simulink model "turbo_controller"  (R2025a)
settings: Solver=FixedStepAuto  StartTime=0.0  StopTime=inf  FixedStep=0.001  RelTol=1e-3
PostLoadFcn:
  | % 自动定位同目录CubeMX文件；不需要外部初始化脚本。
  | codertarget.data.setParameterValue('turbo_controller','STM32CubeMX.ProjectFile',fullfile(fileparts(get_param('turbo_controller','FileName')),'turbo_f407.ioc'));
InitFcn:
  | % 中文说明：按原控制器字段与类型创建三组接口总线；控制参数已内嵌。
  | tc_names=["EValve_Cycle" "EValve_Open" "Eblast_Cycle" "Eblast_Open" "Motor_Cycle" "Motor_Open" "EValve_Enable" "Eblast_Enable" "Motor_Enable" "SWO_Firework" "SWO_BleedAir" "EngineState" "Flag_ECUReset_Clear" "Flag_ECUReset_Save" "Flag_Reset_Enable" "Accelerator" "Nc_dem" "Nc"]; tc_types=["uint16" "uint16" "uint16" "uint16" "uint16" "uint16" "uint8" "uint8" "uint8" "uint8" "uint8" "uint8" "uint8" "uint8" "uint8" "single" "single" "single"];
  | for tc_k=1:numel(tc_names)
  |  tc_e(tc_k)=Simulink.BusElement; tc_e(tc_k).Name=char(tc_names(tc_k)); tc_e(tc_k).DataType=char(tc_types(tc_k));
  | end
  | EngineControl_Out=Simulink.Bus; EngineControl_Out.DataScope='Exported'; EngineControl_Out.Elements=tc_e;
  | clear tc_e tc_names tc_types tc_k
  | tc_names=["savedata1" "savedata2" "savedata3" "savedata4" "savedata5" "savedata6" "savedata7" "savedata8" "savedata9" "savedata10" "savedata11" "savedata12" "savedata13" "savedata14" "savedata15" "savedata16" "savedata17" "savedata18" "savedata19" "savedata20" "savedata21" "savedata22" "savedata23" "savedata24" "savedata25"]; tc_types=["single" "single" "single" "single" "single" "single" "single" "single" "single" "single" "single" "single" "single" "single" "single" "single" "single" "single" "single" "single" "single" "single" "single" "single" "single"];
  | for tc_k=1:numel(tc_names)
  |  tc_e(tc_k)=Simulink.BusElement; tc_e(tc_k).Name=char(tc_names(tc_k)); tc_e(tc_k).DataType=char(tc_types(tc_k));
  | end
  | SaveData_Out=Simulink.Bus; SaveData_Out.DataScope='Exported'; SaveData_Out.Elements=tc_e;
  | clear tc_e tc_names tc_types tc_k
  | tc_names=["senddata1" "senddata2" "senddata3" "senddata4" "senddata5" "senddata6" "senddata7" "senddata8" "senddata9" "senddata10" "senddata11" "senddata12" "senddata13" "senddata14" "senddata15" "senddata16" "senddata17" "senddata18" "senddata19" "senddata20" "senddata21" "senddata22" "senddata23" "senddata24" "senddata25" "senddata26" "senddata27" "senddata28" "senddata29"]; tc_types=["uint8" "uint8" "uint8" "uint8" "uint8" "uint8" "uint8" "uint8" "uint8" "uint8" "uint8" "uint8" "uint8" "uint8" "uint8" "uint8" "uint8" "uint8" "uint8" "uint8" "uint8" "uint8" "uint8" "uint8" "uint8" "uint8" "uint8" "uint8" "uint8"];
  | for tc_k=1:numel(tc_names)
  |  tc_e(tc_k)=Simulink.BusElement; tc_e(tc_k).Name=char(tc_names(tc_k)); tc_e(tc_k).DataType=char(tc_types(tc_k));
  | end
  | SendData_Out=Simulink.Bus; SendData_Out.DataScope='Exported'; SendData_Out.Elements=tc_e;
  | clear tc_e tc_names tc_types tc_k
  | 
  | % 以下为接口中文说明；只设置描述，不改变数值或数据类型。
  | EngineControl_Out.Description='执行控制输出（阀、电机、点火、状态及复位请求）';
  | tc_cn=["EValve_Cycle（主油阀周期计数（每计数2毫秒））" "EValve_Open（主油阀开通计数（每计数2毫秒））" "Eblast_Cycle（副油阀周期计数（每计数2毫秒））" "Eblast_Open（副油阀开通计数（每计数2毫秒））" "Motor_Cycle（起动电机周期计数）" "Motor_Open（起动电机开通计数）" "EValve_Enable（主油阀驱动使能）" "Eblast_Enable（副油阀驱动使能）" "Motor_Enable（起动电机使能）" "SWO_Firework（点火器使能（1开））" "SWO_BleedAir（引气阀使能（1开））" "EngineState（发动机状态）" "Flag_ECUReset_Clear（清除复位恢复状态请求）" "Flag_ECUReset_Save（保存复位恢复数据请求）" "Flag_Reset_Enable（处理器软件复位请求）" "Accelerator（油门／油泵给定控制量）" "Nc_dem（控制目标转速）" "Nc（发动机反馈转速（转每分））"];
  | tc_elements=EngineControl_Out.Elements;
  | for tc_k=1:numel(tc_cn)
  |  tc_elements(tc_k).Description=char(tc_cn(tc_k));
  | end
  | EngineControl_Out.Elements=tc_elements;
  | clear tc_cn tc_elements tc_k
  | SaveData_Out.Description='25项运行记录；字段含义按当前模型数据来源解释';
  | tc_cn=["savedata1（指令回显记录）" "savedata2（入口总温记录（℃））" "savedata3（电源电压记录）" "savedata4（排气温度记录（℃））" "savedata5（标定燃油压力记录）" "savedata6（副油阀占空比记录（％））" "savedata7（主油阀占空比记录（％））" "savedata8（温度修正转速记录）" "savedata9（开关输出及反馈位域）" "savedata10（物理转速记录）" "savedata11（油泵目标给定原始值）" "savedata12（起动电机占空比记录（％））" "savedata13（发动机状态码记录）" "savedata14（故障告警位域记录）" "savedata15（模型记录帧序号）" "savedata16（处理器温度记录（℃））" "savedata17（装订转速记录（沿用旧电源字段名））" "savedata18（导航高度记录）" "savedata19（飞行空速记录）" "savedata20（主阀旧记录位（恒零保留））" "savedata21（第21项保留记录（恒零））" "savedata22（保留记录项22）" "savedata23（保留记录项23）" "savedata24（保留记录项24）" "savedata25（保留记录项25）"];
  | tc_elements=SaveData_Out.Elements;
  | for tc_k=1:numel(tc_cn)
  |  tc_elements(tc_k).Description=char(tc_cn(tc_k));
  | end
  | SaveData_Out.Elements=tc_elements;
  | clear tc_cn tc_elements tc_k
  | SendData_Out.Description='29字段回传及外设命令接口；板端上位机帧只取第3至27字段';
  | tc_cn=["senddata1（回传发送允许标志（不直接上线路））" "senddata2（回传载荷长度25字节）" "senddata3（回传指令回显字节）" "senddata4（总温编码字节（℃＋80））" "senddata5（电源电压编码字节）" "senddata6（排温编码高字节）" "senddata7（排温编码低字节）" "senddata8（燃油压力编码高字节）" "senddata9（燃油压力编码低字节）" "senddata10（副油阀占空比字节（％））" "senddata11（主油阀占空比字节（％））" "senddata12（修正转速编码高字节）" "senddata13（修正转速编码低字节）" "senddata14（驱动及反馈状态位域）" "senddata15（物理转速编码高字节）" "senddata16（物理转速编码低字节）" "senddata17（油泵目标给定高字节（串口二使用））" "senddata18（油泵目标给定低字节（串口二使用））" "senddata19（起动电机占空比命令（串口一使用））" "senddata20（发动机状态码字节）" "senddata21（故障告警位域字节）" "senddata22（帧序号占位（板端另行填写））" "senddata23（处理器温度编码（℃＋50））" "senddata24（控制目标转速编码高字节）" "senddata25（控制目标转速编码低字节）" "senddata26（占位字节（板端改填实测泵速高字节））" "senddata27（占位字节（板端改填实测泵速低字节））" "senddata28（装订转速高字节（本板未发送））" "senddata29（装订转速低字节（本板未发送））"];
  | tc_elements=SendData_Out.Elements;
  | for tc_k=1:numel(tc_cn)
  |  tc_elements(tc_k).Description=char(tc_cn(tc_k));
  | end
  | SendData_Out.Elements=tc_elements;
  | clear tc_cn tc_elements tc_k
  | 
  | 
  | % FRAM模块化事务：接口类型和上电初始状态，随模型保存，无外部初始化文件。
  | clear FM_elements
  | FM_elements(1)=Simulink.BusElement;FM_elements(1).Name='phase';FM_elements(1).DataType='uint8';FM_elements(1).Dimensions=[1 1];FM_elements(1).Description='phase（当前事务阶段）';
  | FM_elements(2)=Simulink.BusElement;FM_elements(2).Name='a';FM_elements(2).DataType='uint8';FM_elements(2).Dimensions=[64 1];FM_elements(2).Description='a（启动时缓存的首区64字节）';
  | FM_elements(3)=Simulink.BusElement;FM_elements(3).Name='active';FM_elements(3).DataType='uint16';FM_elements(3).Dimensions=[1 1];FM_elements(3).Description='active（当前有效记录区地址）';
  | FM_elements(4)=Simulink.BusElement;FM_elements(4).Name='generation';FM_elements(4).DataType='uint32';FM_elements(4).Dimensions=[1 1];FM_elements(4).Description='generation（当前有效记录代号）';
  | FM_elements(5)=Simulink.BusElement;FM_elements(5).Name='record';FM_elements(5).DataType='uint8';FM_elements(5).Dimensions=[64 1];FM_elements(5).Description='record（本次冻结的待写记录）';
  | FM_elements(6)=Simulink.BusElement;FM_elements(6).Name='addr';FM_elements(6).DataType='uint16';FM_elements(6).Dimensions=[1 1];FM_elements(6).Description='addr（本次备用写入地址）';
  | FM_elements(7)=Simulink.BusElement;FM_elements(7).Name='lastSave';FM_elements(7).DataType='single';FM_elements(7).Dimensions=[1 1];FM_elements(7).Description='lastSave（上次开始保存的秒数）';
  | FM_elements(8)=Simulink.BusElement;FM_elements(8).Name='lastState';FM_elements(8).DataType='uint8';FM_elements(8).Dimensions=[1 1];FM_elements(8).Description='lastState（上次保存时的发动机状态）';
  | FM_elements(9)=Simulink.BusElement;FM_elements(9).Name='boot';FM_elements(9).DataType='boolean';FM_elements(9).Dimensions=[1 1];FM_elements(9).Description='boot（启动记录是否允许恢复）';
  | FM_elements(10)=Simulink.BusElement;FM_elements(10).Name='consumed';FM_elements(10).DataType='boolean';FM_elements(10).Dimensions=[1 1];FM_elements(10).Description='consumed（本次启动恢复通知是否已发送）';
  | FM_elements(11)=Simulink.BusElement;FM_elements(11).Name='payload';FM_elements(11).DataType='uint8';FM_elements(11).Dimensions=[20 1];FM_elements(11).Description='payload（当前20字节恢复内容）';
  | ... (+35 lines)
model workspace (MAT data in the model file):
  CRC16_Table_Reference = [0 4129 8258 12387 16516 20645 24774 28903 33032 37161 41290 45419 ... (256 elements, 256x1)]
  PE_Kaer = [0.15402 0.15402 0.12264 0.10076 0.09481 0.07601 0.07111 0.0569 0.05198 0.04926 0.05308 0.04325 ... (13 elements, 1x13)]
  PE_Nr = [21.2982 61.4260372 67.7475458 72.7394382 76.845934 80.6988798 83.8449282 86.6491912 88.9382406 89.178606 91.1938214 93.4068058 ... (13 elements, 1x13)]
  PE_Pump_Translate = 33.5999984741
  PE_RotaSpeed_Translate = 860
  PE_Taer = [0.4939154 0.4939154 0.40780982 0.34066978 0.31622756 0.30405716 0.34300244 0.26785022 0.37393554 0.23914836 0.44563948 0.31044662 ... (13 elements, 1x13)]
  PF_ACCFULLRANGE = 3360
  PF_Flag_ECUReset = 0
  PF_Flag_rx_suc = 1
  PF_Gear_Info = [40000; 45000; 50000; 55000; 57000; 59000; 60000; 61000; 61000; 61000; 61000; 61000]
  PF_K_TiaoJie = 1
  PF_Kpu = 10
  PF_MySet_Rxdata = [0 0 0 0 0 0 0 0 0 0 0 0 ... (50 elements, 50x1)]
  PF_MyUsart1_Rxdata = [0 0 0 0 0 0 0 0 0 0 0 0 ... (50 elements, 50x1)]
  PF_MyUsart2_Rxdata = [0 0 0 0 0 0 0 0 0 0 0 0 ... (50 elements, 50x1)]
  PF_Reset_Information = [0 0 0 0 0 0 0 0 0 0 0 0 ... (20 elements, 20x1)]
  PF_Sensor_X1_T4 = [0 4095]
  PF_Sensor_X2_T4 = [0 1.66666698456]
  PF_Sensor_X3_T4 = [0 504 999 1497 2010 2529 3051 3568 4076 4571 4959]
  PF_Sensor_X_P2 = [0.5 3]
  PF_Sensor_X_Poil = [0.5 3]
  PF_Sensor_X_T1t = [-50 300]
  PF_Sensor_X_Vpower = [0 3]
  PF_Sensor_X_Vpump = [0 3]
  PF_Sensor_Y1_T4 = [0 3]
  PF_Sensor_Y2_T4 = [0 5000]
  PF_Sensor_Y3_T4 = [0 100 200 300 400 500 600 700 800 900 980]
  PF_Sensor_Y_P2 = [0 1000]
  PF_Sensor_Y_Poil = [0 1000]
  PF_Sensor_Y_T1t = [-50 300]
  PF_Sensor_Y_Vpower = [0 33]
  PF_Sensor_Y_Vpump = [0 33]
  PG_CtrlMode_CloseLoop : mpt.Parameter (value not decoded)
  PG_CtrlMode_ManualAcc : mpt.Parameter (value not decoded)
  PG_CtrlMode_Origin : mpt.Parameter (value not decoded)
  PG_CtrlMode_Start : mpt.Parameter (value not decoded)
  PG_CtrlMode_Stop : mpt.Parameter (value not decoded)
  PG_ES_Clp : mpt.Parameter (value not decoded)
  PG_ES_EngStart : mpt.Parameter (value not decoded)
  PG_ES_Manual : mpt.Parameter (value not decoded)
  PG_ES_Origin : mpt.Parameter (value not decoded)
  PG_ES_Stop : mpt.Parameter (value not decoded)
  PG_Instr_BleedAirSet : mpt.Parameter (value not decoded)
  PG_Instr_CloseLoop : mpt.Parameter (value not decoded)
  PG_Instr_ECUReSet : mpt.Parameter (value not decoded)
  PG_Instr_EValveSet : mpt.Parameter (value not decoded)
  PG_Instr_EblastSet : mpt.Parameter (value not decoded)
  PG_Instr_Erase : mpt.Parameter (value not decoded)
  PG_Instr_FireWorkSet : mpt.Parameter (value not decoded)
  PG_Instr_ManualPlus : mpt.Parameter (value not decoded)
  PG_Instr_ManualrReduce : mpt.Parameter (value not decoded)
  PG_Instr_MotorSet : mpt.Parameter (value not decoded)
  PG_Instr_OilSet : mpt.Parameter (value not decoded)
  PG_Instr_SelfCheck : mpt.Parameter (value not decoded)
  PG_Instr_Start : mpt.Parameter (value not decoded)
  PG_Instr_Stop : mpt.Parameter (value not decoded)
  PG_Instr_StopZero : Simulink.Parameter (value not decoded)
  PG_Location_Air : Simulink.Parameter (value not decoded)
  PG_Location_Gnd : Simulink.Parameter (value not decoded)
  PG_ServoCtrlMode_CloseLoop : Simulink.Parameter (value not decoded)
  PG_ServoCtrlMode_CloseLoopMax : Simulink.Parameter (value not decoded)
  PG_ServoCtrlMode_CloseLoopMin : Simulink.Parameter (value not decoded)
  PG_ServoCtrlMode_ManualAcc : Simulink.Parameter (value not decoded)
  PG_ServoCtrlMode_ManualAccMax : Simulink.Parameter (value not decoded)
  PG_ServoCtrlMode_ManualAccMin : Simulink.Parameter (value not decoded)
  PG_SpeedDot_Permit : Simulink.Parameter (value not decoded)
  PL_EngineModel_Actuator = [0 10 100]
  PL_EngineModel_EngineStar_Press_P2 = [1013 1098.4 1099.144828 1099.931034 1103.613793 1162.662069 1143.793103 1131.006897 1123.186207 1117.6 1114 1111.806897 ... (127 elements, 1x127)]
  PL_EngineModel_EngineStar_RotaSpeed = [200 2000 9584 9660 10220 10240 10260 10288 10308 10368 10380 10408 ... (127 elements, 1x127)]
  PL_EngineModel_EngineStar_Temp_Exhaust = [128 129 129.1 130 131 131.1 132 133 134 134.1 135 135.1 ... (127 elements, 1x127)]
  PL_EngineModel_EngineStar_Time = [0.05 0.1 0.15 0.2 0.25 0.3 0.35 0.4 0.45 0.5 0.55 0.6 ... (127 elements, 1x127)]
  PL_EngineModel_IdleAbove_Nr = [0 21.2982 61.4260372 67.7475458 72.7394382 76.845934 80.6988798 83.8449282 86.6491912 88.9382406 89.178606 91.1938214 ... (14 elements, 1x14)]
  PL_EngineModel_IdleAbove_P2r = [0.986923266716 1.57907722675 1.81593881076 1.99358499877 2.23044658278 2.43770046879 2.65482358747 2.84233900814 3.03972366149 3.18776215149 3.25684678016 3.3950160375 ... (14 elements, 1x14)]
  PL_EngineModel_IdleAbove_Tempr = [0.0536001429337 1.07200285867 1.63301768805 1.63659103091 1.66875111667 1.72592460247 1.77595140254 1.86171163123 1.95461854565 2.03323208862 2.03323208862 2.13685903162 ... (14 elements, 1x14)]
  PL_EngineModel_IdleAbove_Ter = [0.42434128 0.42434128 0.42434128 0.30669408 0.23570008 0.22150128 0.1997974 0.23803274 0.16115638 0.24279948 0.13600422 0.31308354 ... (14 elements, 1x14)]
  PL_EngineModel_IdleAbove_Wfr = [0 10.142 23.8337 27.8905 31.9473 36.0041 40.0609 44.1177 48.1745 52.2313 52.7384 56.7952 ... (14 elements, 1x14)]
  PL_EngineModel_Press_P2 = [400 400 400 400 400 400 400 400 400 400]
  PL_EngineModel_Rotaspeed = [0 20000 96400]
  PL_EngineModel_Temp_Exhaust = [500 500 500 500 500 500 500 500 500 500]
  PL_Kaer = [0.1 0.1 0.1 0.1 0.1 0.1]
  PL_Nr = [50 60 70 80 90 100]
  PL_Taer = [0.1 0.1 0.1 0.1 0.1 0.1]
  Sig : Simulink.Signal (value not decoded)
  Ts_ms : Simulink.Parameter (value not decoded)
  false : Simulink.Parameter (value not decoded)
  true : Simulink.Parameter (value not decoded)
symbols that are objects in the model workspace (value not decoded): PG_CtrlMode_CloseLoop, PG_CtrlMode_ManualAcc, PG_CtrlMode_Origin, PG_CtrlMode_Start, PG_CtrlMode_Stop, PG_ES_Clp, PG_ES_EngStart, PG_ES_Manual, PG_ES_Origin, PG_ES_Stop, PG_Instr_BleedAirSet, PG_Instr_CloseLoop, PG_Instr_EblastSet, PG_Instr_ECUReSet, PG_Instr_Erase, PG_Instr_EValveSet, PG_Instr_FireWorkSet, PG_Instr_ManualPlus, PG_Instr_ManualrReduce, PG_Instr_MotorSet, PG_Instr_OilSet, PG_Instr_SelfCheck, PG_Instr_Start, PG_Instr_Stop, PG_Instr_StopZero, PG_ServoCtrlMode_CloseLoop, PG_ServoCtrlMode_CloseLoopMax, PG_ServoCtrlMode_CloseLoopMin, PG_ServoCtrlMode_ManualAcc, PG_ServoCtrlMode_ManualAccMax, PG_ServoCtrlMode_ManualAccMin, Ts_ms
libraries: simulink x97, stm32blockslib x10, stm32f4xxblockslib x8
(part 23 of 26)

== system turbo_controller/BoardInput_输入换算与协议解析/In02_Motor（电机反馈解析）/Receive（逐字节组帧与保持有效结果）_235/Step02_拼帧并保存半帧/Collect（帧头识别与缓存推进）_167/Step04_写入字节或保持原缓存 ==
  note: 第四步：只更新应写的一项，其他内容保留
      |
      | 输入包括旧缓存、本次Byte、候选写入位置和写许可。先将索引取min(候选位置,9)，防止索引超过9项
      | 缓存上界，再用Assignment生成“把这一项换成Byte”的候选数组。
      |
      | 最终选择：写许可为真输出更新数组；写许可为假直接输出旧缓存。即使内部算出了候选更新，只要没
      | 有许可，它也不会成为输出。
      |
      | 例：旧位置为5，本次允许接收，就把第6项换成本字节，其他8项保持；若本字节无效或第二帧头错，
      | 整份缓存保持。缓存里旧的尾部数据并不会每次清零，所以必须配合Complete和后续校验使用，不能只
      | 看数组里有值就当作新帧。
      |
      | 本步骤不保存跨调用记忆。输出回外层的缓存记忆，供下一个字节/下一批数据继续使用。位置更新与
      | 收齐事件在第五步处理。
  输入1_本字节允许写缓存 : Inport
  输入2_上一份候选缓存 : Inport  Port=2
  输入3_候选写入位置 : Inport  Port=3
  输入4_本项字节 : Inport  Port=4
  不允许写则沿用旧缓存 : Switch  Criteria=u2 ~= 0  SaturateOnIntegerOverflow=off  InputSameDT=off
  只替换缓存这一项 : Assignment  DiagnosticForDimensions=Warning  IndexOptions=Index vector (port)  Indices=1  OutputSizes=1
  索引不超过9 : MinMax  Inputs=2
  缓存最大索引9 : Constant  Value=9  OutDataTypeStr=uint16
  输出1_更新后的候选缓存 : Outport
  wires:
  不允许写则沿用旧缓存/1 -> 输出1_更新后的候选缓存/1
  索引不超过9/1 -> 只替换缓存这一项/3
  输入4_本项字节/1 -> 只替换缓存这一项/2
  缓存最大索引9/1 -> 索引不超过9/2
  输入3_候选写入位置/1 -> 索引不超过9/1
  输入2_上一份候选缓存/1 -> 只替换缓存这一项/1, 不允许写则沿用旧缓存/3
  输入1_本字节允许写缓存/1 -> 不允许写则沿用旧缓存/2
  只替换缓存这一项/1 -> 不允许写则沿用旧缓存/1

== system turbo_controller/BoardInput_输入换算与协议解析/In02_Motor（电机反馈解析）/Receive（逐字节组帧与保持有效结果）_235/Step02_拼帧并保存半帧/Collect（帧头识别与缓存推进）_167/Step05_更新收帧位置并报告收齐 ==
  note: 第五步：确定下一次收帧位置，并报告刚收齐
      |
      | 先按收帧阶段选择下一Position：
      | 正在找AA：本字节是AA则到1，否则到0；
      | 正在等55但本字节不匹配：若又是AA则保持1，其他值回0；
      | 正常收数据：未到帧尾就采用Position+1，达到9项后回0，准备找下一帧头。
      | 最后再检查Active：为假时直接保留旧Position，上面的候选变化都不采用。
      |
      | 收齐事件=Active AND 不在等待第一个AA AND 第二帧头没错 AND 达到9项。
      | 因此它只在有效字节刚补上最后一项时为真，不是缓存里有9项就一直为真。位置回0时，完整缓存仍保
      | 留供外层校验。
      |
      | 例：Position=8，有效字节到来，输出Position=0且Complete=true；同样的位置但Active=false，则
      | 输出仍为8且Complete=false。AA、AA、55的序列依次得到位置1、1、2。
      |
      | 本页不验证CRC或累加/异或校验，也不等待下一个20 ms节拍；Complete交外层决定是否接受这条候选
      | 帧。
  输入1_当前字节等于AA : Inport
  输入2_本项字节有效 : Inport  Port=2
  输入3_候选位置达到帧长 : Inport  Port=3
  输入4_候选写入位置 : Inport  Port=4
  输入5_本次之前已收字节数 : Inport  Port=5
  输入6_正在寻找第一个AA : Inport  Port=6
  输入7_第二帧头不匹配 : Inport  Port=7
  AA匹配结果转成0或1 : DataTypeConversion  OutDataTypeStr=uint16  RndMeth=Round
  刚收齐一帧 : Logic  Inputs=4  IconShape=distinctive  AllPortsSameDT=off  OutDataTypeStr=boolean
  已经越过寻找AA阶段 : Logic  Operator=NOT  Inputs=1  IconShape=distinctive  AllPortsSameDT=off  OutDataTypeStr=boolean
  无效字节保持原位置 : Switch  Criteria=u2 ~= 0  SaturateOnIntegerOverflow=off  InputSameDT=off
  满帧回0_未满继续 : Switch  Criteria=u2 ~= 0  SaturateOnIntegerOverflow=off  InputSameDT=off
  第二帧头没有错 : Logic  Operator=NOT  Inputs=1  IconShape=distinctive  AllPortsSameDT=off  OutDataTypeStr=boolean
  第二帧头错则重新找 : Switch  Criteria=u2 ~= 0  SaturateOnIntegerOverflow=off  InputSameDT=off
  起始位置0 : Constant  Value=0  OutDataTypeStr=uint16
  起点只接收AA : Switch  Criteria=u2 ~= 0  SaturateOnIntegerOverflow=off  InputSameDT=off
  输出1_下一次已收字节数 : Outport
  输出2_本字节刚收齐 : Outport  Port=2
  wires:
  输入1_当前字节等于AA/1 -> AA匹配结果转成0或1/1
  输入6_正在寻找第一个AA/1 -> 起点只接收AA/2, 已经越过寻找AA阶段/1
  输入3_候选位置达到帧长/1 -> 刚收齐一帧/4, 满帧回0_未满继续/2
  起始位置0/1 -> 满帧回0_未满继续/1
  输入4_候选写入位置/1 -> 满帧回0_未满继续/3
  AA匹配结果转成0或1/1 -> 第二帧头错则重新找/1, 起点只接收AA/1
  满帧回0_未满继续/1 -> 第二帧头错则重新找/3
  输入7_第二帧头不匹配/1 -> 第二帧头没有错/1, 第二帧头错则重新找/2
  第二帧头错则重新找/1 -> 起点只接收AA/3
  输入2_本项字节有效/1 -> 无效字节保持原位置/2, 刚收齐一帧/1
  已经越过寻找AA阶段/1 -> 刚收齐一帧/2
  第二帧头没有错/1 -> 刚收齐一帧/3
  起点只接收AA/1 -> 无效字节保持原位置/1
  输入5_本次之前已收字节数/1 -> 无效字节保持原位置/3
  刚收齐一帧/1 -> 输出2_本字节刚收齐/1
  无效字节保持原位置/1 -> 输出1_下一次已收字节数/1

== system turbo_controller/BoardInput_输入换算与协议解析/In02_Motor（电机反馈解析）/Receive（逐字节组帧与保持有效结果）_235/Step03_收齐且校验通过才接受/Verify（完整帧校验）_218/CRC16（循环冗余校验）_202 ==
  note: 整段字节如何逐个累积CRC16
      |
      | 这里的输入Bytes是接收帧中由父级Selector选出的数据段。CRC的作用是把整段字节压缩成一个16位检
      | 查值，便于接收方发现传输内容变化。
      |
      | 每帧从初始CRC=uint16(0)开始。循环一次取一个字节，把该字节乘256移到高8位，与旧CRC异或，得到
      | Merged，再交给TableStep执行查表移位。TableStep的输出成为处理下一个字节的旧CRC。
      |
      | 公式第一步是Merged=bitxor(旧CRC,当前字节×256)。整个循环结束后输出最后一次CRC，父级拆成高、
      | 低字节用于比较或发送。For Iterator中的CRC记忆是帧内累积状态，不能理解成跨帧无限累加。
      |
      | 这里用的是CRC16_Table_Reference指定的算法表，不能随意换另一种CRC表或初始值。相同字节、顺序
      | 、表和初值必须得到相同结果，双方才能校验通过。
  Bytes（待校验字节）_172 : Inport  OutDataTypeStr=uint8
  CRC（本帧累计校验值）_174 : UnitDelay  InitialCondition=uint16(0)  SampleTime=-1  HasFrameUpgradeWarning=on
  Cast（数据类型转换）_176 : DataTypeConversion  OutDataTypeStr=uint16  RndMeth=Round
  Constant（常量）_177 : Constant  Value=256  OutDataTypeStr=uint16
  CurrentByte（当前字节）_175 : Selector  InputPortWidth=2  IndexOptions=Index vector (port)  Indices=1  OutputSizes=1
  EachByte（逐字节校验）_173 : ForIterator  ResetStates=reset  IterationLimit=2  IterationVariableDataType=uint32
  HighByte（字节移到高八位）_178 : Product  Inputs=**  SaturateOnIntegerOverflow=on  OutDataTypeStr=Inherit: Same as first input
  MergeByte（并入一个字节）_179 : simulink/Logic and Bit Operations/Bitwise Operator  logicop=XOR  UseBitMask=off  NumInputPorts=2  BitMask=bin2dec('11011001')  BitMaskRealWorld=Stored Integer
      settings: LibrarySourceBlock=|
      | hdlsllib/Logic and Bit
      | Operations/Bitwise
      | Operator
  Store_uint16（按十六位无符号数保存状态）_536668 : DataTypeConversion  Description=为反馈回路显式指定原程序的状态类型，保持原状态更新节拍。  OutDataTypeStr=uint16  RndMeth=Round
  TableStep（查表更新本字节校验） : Subsystem  Description=|
      | CRC16的一个字节怎样查表更新
      | 
      | 父级已经把当前数据字节异或进旧CRC的高8位，形成Merged。本模块把这个16位数拆成“用哪项表”和“保留哪些移位结果”两部分。
      | 
      | 先取高8位：索引=floor(Merged/256)，范围0～255。用它到CRC16_Table_Reference查表；模型Selector按零基索引取值，写成MATLAB数组下标时要用索引+1。
      | 另一条支路把Merged左移一个字节，即乘256，然后只保留低16位：移位值=bitand(uint32(Merged)×256,65535)。
      | 
      | 最后将表值与移位值按位异或：
      | 新CRC=bitxor(表值,移位值)。
      | 
      | 例如Merged=十六进制1234，高8位12用于选表项，左移并截16位后为3400，再与表项异或。宽类型uint32是为了中间计算不先溢出，并不表示输出CRC变成32位。结果回到父级，继续处理下一个数据字节。
  CRC16（本帧校验结果）_201 : Outport
  wires:
  Bytes（待校验字节）_172/1 -> CurrentByte（当前字节）_175/1  "Bytes（待校验字节）"
  CRC（本帧累计校验值）_174/1 -> MergeByte（并入一个字节）_179/1  "CRC（本帧累计校验值）"
  TableStep（查表更新本字节校验）/1(CRC（本字节处理后的校验值）) -> Store_uint16（按十六位无符号数保存状态）_536668/1, CRC16（本帧校验结果）_201/1  "CRC16（查表更新结果）"
  EachByte（逐字节校验）_173/1 -> CurrentByte（当前字节）_175/2  "EachByte（逐字节校验）"
  Constant（常量）_177/1 -> HighByte（字节移到高八位）_178/2  "Constant（常量）"
  CurrentByte（当前字节）_175/1 -> Cast（数据类型转换）_176/1  "CurrentByte（当前字节）"
  Store_uint16（按十六位无符号数保存状态）_536668/1 -> CRC（本帧累计校验值）_174/1
  Cast（数据类型转换）_176/1 -> HighByte（字节移到高八位）_178/1  "Cast（数据类型转换）"
  HighByte（字节移到高八位）_178/1 -> MergeByte（并入一个字节）_179/2  "HighByte（字节移到高八位）"
  MergeByte（并入一个字节）_179/1 -> TableStep（查表更新本字节校验）/1(Merged（旧校验值与当前字节异或后的数）)  "Merged（旧CRC与当前字节合并值）"

== system turbo_controller/BoardInput_输入换算与协议解析/In03_Pump（油泵回包预留校验）/Receive（逐字节组帧与保持有效结果）_353/Step02_拼帧并保存半帧/Collect（帧头识别与缓存推进）_293/Step01_判断收帧阶段与AA55 ==
  note: 第一步：看现在收到哪里，并识别AA、55
      |
      | 只看Position和Byte，不修改缓存，不保存历史。输出三个判断：是否正在找第一个AA、当前字节是否
      | AA、是否发生第二帧头不匹配。
      |
      | Position=0：还没确认帧头，正在找AA。
      | Position=1：已经见到AA，期望下一个是55。
      | Position≥2：头部已确认，后续字节属于帧内数据。
      |
      | AA是十六进制，十进制为170；55是十六进制，十进制为85。判断式：
      | 等待AA=(Position==0)；
      | 字节是AA=(Byte==170)；
      | 第二帧头错=(Position==1) AND (Byte!=85)。
      |
      | 例：Position=1、Byte=AA时，字节是AA和第二帧头错都为真。这并不冲突：它表示没等到55，但可以
      | 把这个AA视作重新找头的机会。是否写入、位置如何调整由后面两步分别处理。
      |
      | 本步骤不检查Active；本字节无效时，后面的写入和位置保持分支会阻止它改变状态。
  输入1_本项字节 : Inport
  输入2_本次之前已收字节数 : Inport  Port=2
  位置为0_等待AA : RelationalOperator  Operator===  OutDataTypeStr=boolean  RndMeth=Simplest  InputSameDT=off
  位置为1_等待55 : RelationalOperator  Operator===  OutDataTypeStr=boolean  RndMeth=Simplest  InputSameDT=off
  已见AA时位置1 : Constant  OutDataTypeStr=uint16
  帧头55_十进制85 : Constant  Value=85  OutDataTypeStr=uint8
  帧头AA_十进制170 : Constant  Value=170  OutDataTypeStr=uint8
  当前字节不是55 : RelationalOperator  Operator=~=  OutDataTypeStr=boolean  RndMeth=Simplest  InputSameDT=off
  当前字节是否AA : RelationalOperator  Operator===  OutDataTypeStr=boolean  RndMeth=Simplest  InputSameDT=off
  等待55却收到其他值 : Logic  IconShape=distinctive  AllPortsSameDT=off  OutDataTypeStr=boolean
  起始位置0 : Constant  Value=0  OutDataTypeStr=uint16
  输出1_当前字节等于AA : Outport
  输出2_正在寻找第一个AA : Outport  Port=2
  输出3_第二帧头不匹配 : Outport  Port=3
  wires:
  等待55却收到其他值/1 -> 输出3_第二帧头不匹配/1
  位置为0_等待AA/1 -> 输出2_正在寻找第一个AA/1
  当前字节是否AA/1 -> 输出1_当前字节等于AA/1
  起始位置0/1 -> 位置为0_等待AA/2
  已见AA时位置1/1 -> 位置为1_等待55/2
  输入2_本次之前已收字节数/1 -> 位置为1_等待55/1, 位置为0_等待AA/1
  帧头55_十进制85/1 -> 当前字节不是55/2
  帧头AA_十进制170/1 -> 当前字节是否AA/2
  输入1_本项字节/1 -> 当前字节是否AA/1, 当前字节不是55/1
  当前字节不是55/1 -> 等待55却收到其他值/2
  位置为1_等待55/1 -> 等待55却收到其他值/1

== system turbo_controller/BoardInput_输入换算与协议解析/In03_Pump（油泵回包预留校验）/Receive（逐字节组帧与保持有效结果）_353/Step02_拼帧并保存半帧/Collect（帧头识别与缓存推进）_293/Step02_判断本字节能否写入 ==
  note: 第二步：决定本字节是否允许写进帧缓存
      |
      | 收帧必须先找到头，所以不是每个字节都写。将第一步的三个判断与Active组合：
      |
      | 允许写入=Active AND [
      |   (正在等AA AND 字节是AA)
      |   OR (不在等AA AND 第二帧头没有错)
      | ]。
      |
      | 分别理解：
      | 还在找AA时，只写AA，其他噪声不进入缓存；
      | 已经见到AA、等待55时，只写正确的55；
      | 头部已经确认后，按顺序接收普通数据，不因数据恰好是AA/55就重新找头；
      | Active为假时，上述条件再合适也不写。
      |
      | 例：已见AA后又来AA，本步骤不把第二个AA写进第2项；后面的重同步位置逻辑仍保留“已见AA”的状
      | 态，继续等55。
      |
      | 输出只是一项布尔写许可，送第四步。它不产生新缓存，也不判断整帧校验。
  输入1_正在寻找第一个AA : Inport
  输入2_当前字节等于AA : Inport  Port=2
  输入3_第二帧头不匹配 : Inport  Port=3
  输入4_本项字节有效 : Inport  Port=4
  字节符合收帧规则 : Logic  Operator=OR  IconShape=distinctive  AllPortsSameDT=off  OutDataTypeStr=boolean
  已经越过寻找AA阶段 : Logic  Operator=NOT  Inputs=1  IconShape=distinctive  AllPortsSameDT=off  OutDataTypeStr=boolean
  已过起点且第二帧头没错 : Logic  IconShape=distinctive  AllPortsSameDT=off  OutDataTypeStr=boolean
  本字节有效且允许写入 : Logic  IconShape=distinctive  AllPortsSameDT=off  OutDataTypeStr=boolean
  第二帧头没有错 : Logic  Operator=NOT  Inputs=1  IconShape=distinctive  AllPortsSameDT=off  OutDataTypeStr=boolean
  起点遇到AA : Logic  IconShape=distinctive  AllPortsSameDT=off  OutDataTypeStr=boolean
  输出1_本字节允许写缓存 : Outport
  wires:
  本字节有效且允许写入/1 -> 输出1_本字节允许写缓存/1
  字节符合收帧规则/1 -> 本字节有效且允许写入/2
  输入4_本项字节有效/1 -> 本字节有效且允许写入/1
  输入3_第二帧头不匹配/1 -> 第二帧头没有错/1
  已过起点且第二帧头没错/1 -> 字节符合收帧规则/2
  起点遇到AA/1 -> 字节符合收帧规则/1
  第二帧头没有错/1 -> 已过起点且第二帧头没错/2
  已经越过寻找AA阶段/1 -> 已过起点且第二帧头没错/1
  输入2_当前字节等于AA/1 -> 起点遇到AA/2
  输入1_正在寻找第一个AA/1 -> 已经越过寻找AA阶段/1, 起点遇到AA/1

== system turbo_controller/BoardInput_输入换算与协议解析/In03_Pump（油泵回包预留校验）/Receive（逐字节组帧与保持有效结果）_353/Step02_拼帧并保存半帧/Collect（帧头识别与缓存推进）_293/Step03_计算写入位置与是否满帧 ==
  note: 第三步：算本次写到第几项，并判断是否到帧尾
      |
      | Position表示本次之前已接收多少项。本次候选写入位置=Position+1；帧长度固定为22，达到帧尾=(
      | 候选写入位置==22)。
      |
      | 例如Position=0时，候选位置是1，AA应写到第1项；Position=1时，55应写到第2项；Position=21时，
      | 本次候选位置是22，这是最后一项。
      |
      | 注意这里算的是“候选位置”：即使Active为假，仍可计算Position+1，但第四、第五步会保持缓存和
      | 位置。不能仅因候选位置等于22就认定收到新帧。
      |
      | 候选位置送第四步写缓存；它及“达到帧尾”标志也送第五步，决定继续推进还是收齐后回0。本处不
      | 保存Position，也不清空缓存。
  输入1_本次之前已收字节数 : Inport
  候选位置是否到帧尾 : RelationalOperator  Operator===  OutDataTypeStr=boolean  RndMeth=Simplest  InputSameDT=off
  固定帧长22 : Constant  Value=22  OutDataTypeStr=uint16
  本次候选位置加一 : Sum  SaturateOnIntegerOverflow=on  OutDataTypeStr=Inherit: Same as first input
  每次推进1项 : Constant  OutDataTypeStr=uint16
  输出1_候选位置达到帧长 : Outport
  输出2_候选写入位置 : Outport  Port=2
  wires:
  候选位置是否到帧尾/1 -> 输出1_候选位置达到帧长/1
  每次推进1项/1 -> 本次候选位置加一/2
  输入1_本次之前已收字节数/1 -> 本次候选位置加一/1
  固定帧长22/1 -> 候选位置是否到帧尾/2
  本次候选位置加一/1 -> 候选位置是否到帧尾/1, 输出2_候选写入位置/1

== system turbo_controller/BoardInput_输入换算与协议解析/In03_Pump（油泵回包预留校验）/Receive（逐字节组帧与保持有效结果）_353/Step02_拼帧并保存半帧/Collect（帧头识别与缓存推进）_293/Step04_写入字节或保持原缓存 ==
  note: 第四步：只更新应写的一项，其他内容保留
      |
      | 输入包括旧缓存、本次Byte、候选写入位置和写许可。先将索引取min(候选位置,22)，防止索引超过22
      | 项缓存上界，再用Assignment生成“把这一项换成Byte”的候选数组。
      |
      | 最终选择：写许可为真输出更新数组；写许可为假直接输出旧缓存。即使内部算出了候选更新，只要没
      | 有许可，它也不会成为输出。
      |
      | 例：旧位置为5，本次允许接收，就把第6项换成本字节，其他21项保持；若本字节无效或第二帧头错，
      | 整份缓存保持。缓存里旧的尾部数据并不会每次清零，所以必须配合Complete和后续校验使用，不能只
      | 看数组里有值就当作新帧。
      |
      | 本步骤不保存跨调用记忆。输出回外层的缓存记忆，供下一个字节/下一批数据继续使用。位置更新与
      | 收齐事件在第五步处理。
  输入1_本字节允许写缓存 : Inport
  输入2_上一份候选缓存 : Inport  Port=2
  输入3_候选写入位置 : Inport  Port=3
  输入4_本项字节 : Inport  Port=4
  不允许写则沿用旧缓存 : Switch  Criteria=u2 ~= 0  SaturateOnIntegerOverflow=off  InputSameDT=off
  只替换缓存这一项 : Assignment  DiagnosticForDimensions=Warning  IndexOptions=Index vector (port)  Indices=1  OutputSizes=1
  索引不超过22 : MinMax  Inputs=2
  缓存最大索引22 : Constant  Value=22  OutDataTypeStr=uint16
  输出1_更新后的候选缓存 : Outport
  wires:
  不允许写则沿用旧缓存/1 -> 输出1_更新后的候选缓存/1
  索引不超过22/1 -> 只替换缓存这一项/3
  输入4_本项字节/1 -> 只替换缓存这一项/2
  缓存最大索引22/1 -> 索引不超过22/2
  输入3_候选写入位置/1 -> 索引不超过22/1
  输入2_上一份候选缓存/1 -> 只替换缓存这一项/1, 不允许写则沿用旧缓存/3
  输入1_本字节允许写缓存/1 -> 不允许写则沿用旧缓存/2
  只替换缓存这一项/1 -> 不允许写则沿用旧缓存/1

== system turbo_controller/BoardInput_输入换算与协议解析/In03_Pump（油泵回包预留校验）/Receive（逐字节组帧与保持有效结果）_353/Step02_拼帧并保存半帧/Collect（帧头识别与缓存推进）_293/Step05_更新收帧位置并报告收齐 ==
  note: 第五步：确定下一次收帧位置，并报告刚收齐
      |
      | 先按收帧阶段选择下一Position：
      | 正在找AA：本字节是AA则到1，否则到0；
      | 正在等55但本字节不匹配：若又是AA则保持1，其他值回0；
      | 正常收数据：未到帧尾就采用Position+1，达到22项后回0，准备找下一帧头。
      | 最后再检查Active：为假时直接保留旧Position，上面的候选变化都不采用。
      |
      | 收齐事件=Active AND 不在等待第一个AA AND 第二帧头没错 AND 达到22项。
      | 因此它只在有效字节刚补上最后一项时为真，不是缓存里有22项就一直为真。位置回0时，完整缓存仍
      | 保留供外层校验。
      |
      | 例：Position=21，有效字节到来，输出Position=0且Complete=true；同样的位置但Active=false，则
      | 输出仍为21且Complete=false。AA、AA、55的序列依次得到位置1、1、2。
      |
      | 本页不验证CRC或累加/异或校验，也不等待下一个20 ms节拍；Complete交外层决定是否接受这条候选
      | 帧。
  输入1_当前字节等于AA : Inport
  输入2_本项字节有效 : Inport  Port=2
  输入3_候选位置达到帧长 : Inport  Port=3
  输入4_候选写入位置 : Inport  Port=4
  输入5_本次之前已收字节数 : Inport  Port=5
  输入6_正在寻找第一个AA : Inport  Port=6
  输入7_第二帧头不匹配 : Inport  Port=7
  AA匹配结果转成0或1 : DataTypeConversion  OutDataTypeStr=uint16  RndMeth=Round
  刚收齐一帧 : Logic  Inputs=4  IconShape=distinctive  AllPortsSameDT=off  OutDataTypeStr=boolean
  已经越过寻找AA阶段 : Logic  Operator=NOT  Inputs=1  IconShape=distinctive  AllPortsSameDT=off  OutDataTypeStr=boolean
  无效字节保持原位置 : Switch  Criteria=u2 ~= 0  SaturateOnIntegerOverflow=off  InputSameDT=off
  满帧回0_未满继续 : Switch  Criteria=u2 ~= 0  SaturateOnIntegerOverflow=off  InputSameDT=off
  第二帧头没有错 : Logic  Operator=NOT  Inputs=1  IconShape=distinctive  AllPortsSameDT=off  OutDataTypeStr=boolean
  第二帧头错则重新找 : Switch  Criteria=u2 ~= 0  SaturateOnIntegerOverflow=off  InputSameDT=off
  起始位置0 : Constant  Value=0  OutDataTypeStr=uint16
  起点只接收AA : Switch  Criteria=u2 ~= 0  SaturateOnIntegerOverflow=off  InputSameDT=off
  输出1_下一次已收字节数 : Outport
  输出2_本字节刚收齐 : Outport  Port=2
  wires:
  刚收齐一帧/1 -> 输出2_本字节刚收齐/1
  无效字节保持原位置/1 -> 输出1_下一次已收字节数/1
  第二帧头错则重新找/1 -> 起点只接收AA/3
  满帧回0_未满继续/1 -> 第二帧头错则重新找/3
  AA匹配结果转成0或1/1 -> 第二帧头错则重新找/1, 起点只接收AA/1
  输入7_第二帧头不匹配/1 -> 第二帧头没有错/1, 第二帧头错则重新找/2
  输入6_正在寻找第一个AA/1 -> 已经越过寻找AA阶段/1, 起点只接收AA/2
  输入5_本次之前已收字节数/1 -> 无效字节保持原位置/3
  起点只接收AA/1 -> 无效字节保持原位置/1
  输入4_候选写入位置/1 -> 满帧回0_未满继续/3
  起始位置0/1 -> 满帧回0_未满继续/1
  输入3_候选位置达到帧长/1 -> 满帧回0_未满继续/2, 刚收齐一帧/4
  第二帧头没有错/1 -> 刚收齐一帧/3
  已经越过寻找AA阶段/1 -> 刚收齐一帧/2
  输入2_本项字节有效/1 -> 无效字节保持原位置/2, 刚收齐一帧/1
  输入1_当前字节等于AA/1 -> AA匹配结果转成0或1/1

== system turbo_controller/BoardInput_输入换算与协议解析/In03_Pump（油泵回包预留校验）/Receive（逐字节组帧与保持有效结果）_353/Step03_收齐且校验通过才接受/Verify（完整帧校验）_344/CRC16（循环冗余校验）_328 ==
  note: 整段字节如何逐个累积CRC16
      |
      | 这里的输入Bytes是接收帧中由父级Selector选出的数据段。CRC的作用是把整段字节压缩成一个16位检
      | 查值，便于接收方发现传输内容变化。
      |
      | 每帧从初始CRC=uint16(0)开始。循环一次取一个字节，把该字节乘256移到高8位，与旧CRC异或，得到
      | Merged，再交给TableStep执行查表移位。TableStep的输出成为处理下一个字节的旧CRC。
      |
      | 公式第一步是Merged=bitxor(旧CRC,当前字节×256)。整个循环结束后输出最后一次CRC，父级拆成高、
      | 低字节用于比较或发送。For Iterator中的CRC记忆是帧内累积状态，不能理解成跨帧无限累加。
      |
      | 这里用的是CRC16_Table_Reference指定的算法表，不能随意换另一种CRC表或初始值。相同字节、顺序
      | 、表和初值必须得到相同结果，双方才能校验通过。
  note: 【中文学习说明：CRC16查表法】
      | 一、大白话：把逐位算出的答案预先放进表里。
      | 收到每个字节后，用旧校验值和当前字节算一个表下标，
      | 直接查出结果，再与旧值左移一个字节后的部分异或。
      | 每字节只查一次表，不再进行8次逐位循环。
      |
      | 二、本模块一次处理15个数据字节。
      | 每帧校验值从0开始；逐字节循环仍按输入顺序执行。
      | 先将当前字节放到高八位，与旧CRC异或，
      | 再交给TableStep（查表更新）算出新CRC，
      | 记住新CRC后处理下一个字节，最后输出16位结果。
      |
      | 三、和参考工程逐项对应。
      | 参考写法：index=((旧CRC>>8) XOR 当前字节) AND 255。
      | 新CRC=表[index] XOR ((旧CRC<<8) AND 65535)。
      | 本图先合并字节再取高八位，得到完全相同的index。
      | 表为参考工程crc.c中的原始256项uint16数据，
      | 保存在模型工作区CRC16_Table_Reference中，
      | 所有CRC16模块使用同一份表，无需额外源文件。
      |
      | 四、协议规则没有改变。
      | 初值0、多项式0x1021、高位先处理、不作末尾异或。
      | 校验范围由外层选取，帧头和帧尾校验字节不随意加入。
      | 输出仍由外层拆成高、低字节，高字节在前。
      | 这里只计算CRC，是否采纳数据由外层校验比较决定。
      |
      | 五、记忆与循环要分清。
      | 外层逐字节循环在一次调用内处理整段数据，
      | 并非每处理一字节就等待一个采样周期。
      | CRC记忆块传递同一帧中上一个字节的结果；
      | 每次重新计算一帧时从0开始，不串用上一帧的结果。
      | 查表能发现传输错误，不能修复数据，也不是加密。
  Bytes（待校验字节）_298 : Inport  OutDataTypeStr=uint8
  CRC（本帧累计校验值）_300 : UnitDelay  InitialCondition=uint16(0)  SampleTime=-1  HasFrameUpgradeWarning=on
  Cast（数据类型转换）_302 : DataTypeConversion  OutDataTypeStr=uint16  RndMeth=Round
  Constant（常量）_303 : Constant  Value=256  OutDataTypeStr=uint16
  CurrentByte（当前字节）_301 : Selector  InputPortWidth=15  IndexOptions=Index vector (port)  Indices=1  OutputSizes=1
  EachByte（逐字节校验）_299 : ForIterator  ResetStates=reset  IterationLimit=15  IterationVariableDataType=uint32
  HighByte（字节移到高八位）_304 : Product  Inputs=**  SaturateOnIntegerOverflow=on  OutDataTypeStr=Inherit: Same as first input
  MergeByte（并入一个字节）_305 : simulink/Logic and Bit Operations/Bitwise Operator  logicop=XOR  UseBitMask=off  NumInputPorts=2  BitMask=bin2dec('11011001')  BitMaskRealWorld=Stored Integer
      settings: LibrarySourceBlock=|
      | hdlsllib/Logic and Bit
      | Operations/Bitwise
      | Operator
  Store_uint16（按十六位无符号数保存状态）_536787 : DataTypeConversion  Description=为反馈回路显式指定原程序的状态类型，保持原状态更新节拍。  OutDataTypeStr=uint16  RndMeth=Round
  TableStep（查表更新本字节校验） : Subsystem  Description=|
      | CRC16的一个字节怎样查表更新
      | 
      | 父级已经把当前数据字节异或进旧CRC的高8位，形成Merged。本模块把这个16位数拆成“用哪项表”和“保留哪些移位结果”两部分。
      | 
      | 先取高8位：索引=floor(Merged/256)，范围0～255。用它到CRC16_Table_Reference查表；模型Selector按零基索引取值，写成MATLAB数组下标时要用索引+1。
      | 另一条支路把Merged左移一个字节，即乘256，然后只保留低16位：移位值=bitand(uint32(Merged)×256,65535)。
      | 
      | 最后将表值与移位值按位异或：
      | 新CRC=bitxor(表值,移位值)。
      | 
      | 例如Merged=十六进制1234，高8位12用于选表项，左移并截16位后为3400，再与表项异或。宽类型uint32是为了中间计算不先溢出，并不表示输出CRC变成32位。结果回到父级，继续处理下一个数据字节。
  CRC16（本帧校验结果）_327 : Outport
  wires:
  Store_uint16（按十六位无符号数保存状态）_536787/1 -> CRC（本帧累计校验值）_300/1
  CRC（本帧累计校验值）_300/1 -> MergeByte（并入一个字节）_305/1  "CRC（本帧累计校验值）"
  HighByte（字节移到高八位）_304/1 -> MergeByte（并入一个字节）_305/2  "HighByte（字节移到高八位）"
  MergeByte（并入一个字节）_305/1 -> TableStep（查表更新本字节校验）/1(Merged（旧校验值与当前字节异或后的数）)  "Merged（旧CRC与当前字节合并值）"
  TableStep（查表更新本字节校验）/1(CRC（本字节处理后的校验值）) -> Store_uint16（按十六位无符号数保存状态）_536787/1, CRC16（本帧校验结果）_327/1  "CRC16（查表更新结果）"
  Bytes（待校验字节）_298/1 -> CurrentByte（当前字节）_301/1  "Bytes（待校验字节）"
  EachByte（逐字节校验）_299/1 -> CurrentByte（当前字节）_301/2  "EachByte（逐字节校验）"
  CurrentByte（当前字节）_301/1 -> Cast（数据类型转换）_302/1  "CurrentByte（当前字节）"
  Cast（数据类型转换）_302/1 -> HighByte（字节移到高八位）_304/1  "Cast（数据类型转换）"
  Constant（常量）_303/1 -> HighByte（字节移到高八位）_304/2  "Constant（常量）"

== system turbo_controller/BoardOutput_串口封装与阀门时序/Out01_Pump（泵反馈解析与滤波）/Receive（逐字节组帧与保持有效结果）_680/Step02_拼帧并保存半帧/Collect（帧头识别与缓存推进）_611/Step01_判断收帧阶段与AA55 ==
  note: 第一步：看现在收到哪里，并识别AA、55
      |
      | 只看Position和Byte，不修改缓存，不保存历史。输出三个判断：是否正在找第一个AA、当前字节是否
      | AA、是否发生第二帧头不匹配。
      |
      | Position=0：还没确认帧头，正在找AA。
      | Position=1：已经见到AA，期望下一个是55。
      | Position≥2：头部已确认，后续字节属于帧内数据。
      |
      | AA是十六进制，十进制为170；55是十六进制，十进制为85。判断式：
      | 等待AA=(Position==0)；
      | 字节是AA=(Byte==170)；
      | 第二帧头错=(Position==1) AND (Byte!=85)。
      |
      | 例：Position=1、Byte=AA时，字节是AA和第二帧头错都为真。这并不冲突：它表示没等到55，但可以
      | 把这个AA视作重新找头的机会。是否写入、位置如何调整由后面两步分别处理。
      |
      | 本步骤不检查Active；本字节无效时，后面的写入和位置保持分支会阻止它改变状态。
  输入1_本项字节 : Inport
  输入2_本次之前已收字节数 : Inport  Port=2
  位置为0_等待AA : RelationalOperator  Operator===  OutDataTypeStr=boolean  RndMeth=Simplest  InputSameDT=off
  位置为1_等待55 : RelationalOperator  Operator===  OutDataTypeStr=boolean  RndMeth=Simplest  InputSameDT=off
  已见AA时位置1 : Constant  OutDataTypeStr=uint16
  帧头55_十进制85 : Constant  Value=85  OutDataTypeStr=uint8
  帧头AA_十进制170 : Constant  Value=170  OutDataTypeStr=uint8
  当前字节不是55 : RelationalOperator  Operator=~=  OutDataTypeStr=boolean  RndMeth=Simplest  InputSameDT=off
  当前字节是否AA : RelationalOperator  Operator===  OutDataTypeStr=boolean  RndMeth=Simplest  InputSameDT=off
  等待55却收到其他值 : Logic  IconShape=distinctive  AllPortsSameDT=off  OutDataTypeStr=boolean
  起始位置0 : Constant  Value=0  OutDataTypeStr=uint16
  输出1_当前字节等于AA : Outport
  输出2_正在寻找第一个AA : Outport  Port=2
  输出3_第二帧头不匹配 : Outport  Port=3
  wires:
  等待55却收到其他值/1 -> 输出3_第二帧头不匹配/1
  位置为0_等待AA/1 -> 输出2_正在寻找第一个AA/1
  当前字节是否AA/1 -> 输出1_当前字节等于AA/1
  起始位置0/1 -> 位置为0_等待AA/2
  已见AA时位置1/1 -> 位置为1_等待55/2
  输入2_本次之前已收字节数/1 -> 位置为1_等待55/1, 位置为0_等待AA/1
  帧头55_十进制85/1 -> 当前字节不是55/2
  帧头AA_十进制170/1 -> 当前字节是否AA/2
  输入1_本项字节/1 -> 当前字节是否AA/1, 当前字节不是55/1
  当前字节不是55/1 -> 等待55却收到其他值/2
  位置为1_等待55/1 -> 等待55却收到其他值/1

== system turbo_controller/BoardOutput_串口封装与阀门时序/Out01_Pump（泵反馈解析与滤波）/Receive（逐字节组帧与保持有效结果）_680/Step02_拼帧并保存半帧/Collect（帧头识别与缓存推进）_611/Step02_判断本字节能否写入 ==
  note: 第二步：决定本字节是否允许写进帧缓存
      |
      | 收帧必须先找到头，所以不是每个字节都写。将第一步的三个判断与Active组合：
      |
      | 允许写入=Active AND [
      |   (正在等AA AND 字节是AA)
      |   OR (不在等AA AND 第二帧头没有错)
      | ]。
      |
      | 分别理解：
      | 还在找AA时，只写AA，其他噪声不进入缓存；
      | 已经见到AA、等待55时，只写正确的55；
      | 头部已经确认后，按顺序接收普通数据，不因数据恰好是AA/55就重新找头；
      | Active为假时，上述条件再合适也不写。
      |
      | 例：已见AA后又来AA，本步骤不把第二个AA写进第2项；后面的重同步位置逻辑仍保留“已见AA”的状
      | 态，继续等55。
      |
      | 输出只是一项布尔写许可，送第四步。它不产生新缓存，也不判断整帧校验。
  输入1_正在寻找第一个AA : Inport
  输入2_当前字节等于AA : Inport  Port=2
  输入3_第二帧头不匹配 : Inport  Port=3
  输入4_本项字节有效 : Inport  Port=4
  字节符合收帧规则 : Logic  Operator=OR  IconShape=distinctive  AllPortsSameDT=off  OutDataTypeStr=boolean
  已经越过寻找AA阶段 : Logic  Operator=NOT  Inputs=1  IconShape=distinctive  AllPortsSameDT=off  OutDataTypeStr=boolean
  已过起点且第二帧头没错 : Logic  IconShape=distinctive  AllPortsSameDT=off  OutDataTypeStr=boolean
  本字节有效且允许写入 : Logic  IconShape=distinctive  AllPortsSameDT=off  OutDataTypeStr=boolean
  第二帧头没有错 : Logic  Operator=NOT  Inputs=1  IconShape=distinctive  AllPortsSameDT=off  OutDataTypeStr=boolean
  起点遇到AA : Logic  IconShape=distinctive  AllPortsSameDT=off  OutDataTypeStr=boolean
  输出1_本字节允许写缓存 : Outport
  wires:
  本字节有效且允许写入/1 -> 输出1_本字节允许写缓存/1
  字节符合收帧规则/1 -> 本字节有效且允许写入/2
  输入4_本项字节有效/1 -> 本字节有效且允许写入/1
  输入3_第二帧头不匹配/1 -> 第二帧头没有错/1
  已过起点且第二帧头没错/1 -> 字节符合收帧规则/2
  起点遇到AA/1 -> 字节符合收帧规则/1
  第二帧头没有错/1 -> 已过起点且第二帧头没错/2
  已经越过寻找AA阶段/1 -> 已过起点且第二帧头没错/1
  输入2_当前字节等于AA/1 -> 起点遇到AA/2
  输入1_正在寻找第一个AA/1 -> 起点遇到AA/1, 已经越过寻找AA阶段/1

== system turbo_controller/BoardOutput_串口封装与阀门时序/Out01_Pump（泵反馈解析与滤波）/Receive（逐字节组帧与保持有效结果）_680/Step02_拼帧并保存半帧/Collect（帧头识别与缓存推进）_611/Step03_计算写入位置与是否满帧 ==
  note: 第三步：算本次写到第几项，并判断是否到帧尾
      |
      | Position表示本次之前已接收多少项。本次候选写入位置=Position+1；帧长度固定为22，达到帧尾=(
      | 候选写入位置==22)。
      |
      | 例如Position=0时，候选位置是1，AA应写到第1项；Position=1时，55应写到第2项；Position=21时，
      | 本次候选位置是22，这是最后一项。
      |
      | 注意这里算的是“候选位置”：即使Active为假，仍可计算Position+1，但第四、第五步会保持缓存和
      | 位置。不能仅因候选位置等于22就认定收到新帧。
      |
      | 候选位置送第四步写缓存；它及“达到帧尾”标志也送第五步，决定继续推进还是收齐后回0。本处不
      | 保存Position，也不清空缓存。
  输入1_本次之前已收字节数 : Inport
  候选位置是否到帧尾 : RelationalOperator  Operator===  OutDataTypeStr=boolean  RndMeth=Simplest  InputSameDT=off
  固定帧长22 : Constant  Value=22  OutDataTypeStr=uint16
  本次候选位置加一 : Sum  SaturateOnIntegerOverflow=on  OutDataTypeStr=Inherit: Same as first input
  每次推进1项 : Constant  OutDataTypeStr=uint16
  输出1_候选位置达到帧长 : Outport
  输出2_候选写入位置 : Outport  Port=2
  wires:
  候选位置是否到帧尾/1 -> 输出1_候选位置达到帧长/1
  每次推进1项/1 -> 本次候选位置加一/2
  输入1_本次之前已收字节数/1 -> 本次候选位置加一/1
  固定帧长22/1 -> 候选位置是否到帧尾/2
  本次候选位置加一/1 -> 候选位置是否到帧尾/1, 输出2_候选写入位置/1

== system turbo_controller/BoardOutput_串口封装与阀门时序/Out01_Pump（泵反馈解析与滤波）/Receive（逐字节组帧与保持有效结果）_680/Step02_拼帧并保存半帧/Collect（帧头识别与缓存推进）_611/Step04_写入字节或保持原缓存 ==
  note: 第四步：只更新应写的一项，其他内容保留
      |
      | 输入包括旧缓存、本次Byte、候选写入位置和写许可。先将索引取min(候选位置,22)，防止索引超过22
      | 项缓存上界，再用Assignment生成“把这一项换成Byte”的候选数组。
      |
      | 最终选择：写许可为真输出更新数组；写许可为假直接输出旧缓存。即使内部算出了候选更新，只要没
      | 有许可，它也不会成为输出。
      |
      | 例：旧位置为5，本次允许接收，就把第6项换成本字节，其他21项保持；若本字节无效或第二帧头错，
      | 整份缓存保持。缓存里旧的尾部数据并不会每次清零，所以必须配合Complete和后续校验使用，不能只
      | 看数组里有值就当作新帧。
      |
      | 本步骤不保存跨调用记忆。输出回外层的缓存记忆，供下一个字节/下一批数据继续使用。位置更新与
      | 收齐事件在第五步处理。
  输入1_本字节允许写缓存 : Inport
  输入2_上一份候选缓存 : Inport  Port=2
  输入3_候选写入位置 : Inport  Port=3
  输入4_本项字节 : Inport  Port=4
  不允许写则沿用旧缓存 : Switch  Criteria=u2 ~= 0  SaturateOnIntegerOverflow=off  InputSameDT=off
  只替换缓存这一项 : Assignment  DiagnosticForDimensions=Warning  IndexOptions=Index vector (port)  Indices=1  OutputSizes=1
  索引不超过22 : MinMax  Inputs=2
  缓存最大索引22 : Constant  Value=22  OutDataTypeStr=uint16
  输出1_更新后的候选缓存 : Outport
  wires:
  不允许写则沿用旧缓存/1 -> 输出1_更新后的候选缓存/1
  索引不超过22/1 -> 只替换缓存这一项/3
  输入4_本项字节/1 -> 只替换缓存这一项/2
  缓存最大索引22/1 -> 索引不超过22/2
  输入3_候选写入位置/1 -> 索引不超过22/1
  输入2_上一份候选缓存/1 -> 只替换缓存这一项/1, 不允许写则沿用旧缓存/3
  输入1_本字节允许写缓存/1 -> 不允许写则沿用旧缓存/2
  只替换缓存这一项/1 -> 不允许写则沿用旧缓存/1

== system turbo_controller/BoardOutput_串口封装与阀门时序/Out01_Pump（泵反馈解析与滤波）/Receive（逐字节组帧与保持有效结果）_680/Step02_拼帧并保存半帧/Collect（帧头识别与缓存推进）_611/Step05_更新收帧位置并报告收齐 ==
  note: 第五步：确定下一次收帧位置，并报告刚收齐
      |
      | 先按收帧阶段选择下一Position：
      | 正在找AA：本字节是AA则到1，否则到0；
      | 正在等55但本字节不匹配：若又是AA则保持1，其他值回0；
      | 正常收数据：未到帧尾就采用Position+1，达到22项后回0，准备找下一帧头。
      | 最后再检查Active：为假时直接保留旧Position，上面的候选变化都不采用。
      |
      | 收齐事件=Active AND 不在等待第一个AA AND 第二帧头没错 AND 达到22项。
      | 因此它只在有效字节刚补上最后一项时为真，不是缓存里有22项就一直为真。位置回0时，完整缓存仍
      | 保留供外层校验。
      |
      | 例：Position=21，有效字节到来，输出Position=0且Complete=true；同样的位置但Active=false，则
      | 输出仍为21且Complete=false。AA、AA、55的序列依次得到位置1、1、2。
      |
      | 本页不验证CRC或累加/异或校验，也不等待下一个20 ms节拍；Complete交外层决定是否接受这条候选
      | 帧。
  输入1_当前字节等于AA : Inport
  输入2_本项字节有效 : Inport  Port=2
  输入3_候选位置达到帧长 : Inport  Port=3
  输入4_候选写入位置 : Inport  Port=4
  输入5_本次之前已收字节数 : Inport  Port=5
  输入6_正在寻找第一个AA : Inport  Port=6
  输入7_第二帧头不匹配 : Inport  Port=7
  AA匹配结果转成0或1 : DataTypeConversion  OutDataTypeStr=uint16  RndMeth=Round
  刚收齐一帧 : Logic  Inputs=4  IconShape=distinctive  AllPortsSameDT=off  OutDataTypeStr=boolean
  已经越过寻找AA阶段 : Logic  Operator=NOT  Inputs=1  IconShape=distinctive  AllPortsSameDT=off  OutDataTypeStr=boolean
  无效字节保持原位置 : Switch  Criteria=u2 ~= 0  SaturateOnIntegerOverflow=off  InputSameDT=off
  满帧回0_未满继续 : Switch  Criteria=u2 ~= 0  SaturateOnIntegerOverflow=off  InputSameDT=off
  第二帧头没有错 : Logic  Operator=NOT  Inputs=1  IconShape=distinctive  AllPortsSameDT=off  OutDataTypeStr=boolean
  第二帧头错则重新找 : Switch  Criteria=u2 ~= 0  SaturateOnIntegerOverflow=off  InputSameDT=off
  起始位置0 : Constant  Value=0  OutDataTypeStr=uint16
  起点只接收AA : Switch  Criteria=u2 ~= 0  SaturateOnIntegerOverflow=off  InputSameDT=off
  输出1_下一次已收字节数 : Outport
  输出2_本字节刚收齐 : Outport  Port=2
  wires:
  刚收齐一帧/1 -> 输出2_本字节刚收齐/1
  无效字节保持原位置/1 -> 输出1_下一次已收字节数/1
  第二帧头错则重新找/1 -> 起点只接收AA/3
  满帧回0_未满继续/1 -> 第二帧头错则重新找/3
  AA匹配结果转成0或1/1 -> 第二帧头错则重新找/1, 起点只接收AA/1
  输入7_第二帧头不匹配/1 -> 第二帧头没有错/1, 第二帧头错则重新找/2
  输入6_正在寻找第一个AA/1 -> 已经越过寻找AA阶段/1, 起点只接收AA/2
  输入5_本次之前已收字节数/1 -> 无效字节保持原位置/3
  起点只接收AA/1 -> 无效字节保持原位置/1
  输入4_候选写入位置/1 -> 满帧回0_未满继续/3
  起始位置0/1 -> 满帧回0_未满继续/1
  输入3_候选位置达到帧长/1 -> 满帧回0_未满继续/2, 刚收齐一帧/4
  第二帧头没有错/1 -> 刚收齐一帧/3
  已经越过寻找AA阶段/1 -> 刚收齐一帧/2
  输入2_本项字节有效/1 -> 无效字节保持原位置/2, 刚收齐一帧/1
  输入1_当前字节等于AA/1 -> AA匹配结果转成0或1/1

== system turbo_controller/BoardOutput_串口封装与阀门时序/Out01_Pump（泵反馈解析与滤波）/Receive（逐字节组帧与保持有效结果）_680/Step03_收齐且校验通过才接受/Verify（完整帧校验）_662/CRC16（循环冗余校验）_646 ==
  note: 整段字节如何逐个累积CRC16
      |
      | 这里的输入Bytes是接收帧中由父级Selector选出的数据段。CRC的作用是把整段字节压缩成一个16位检
      | 查值，便于接收方发现传输内容变化。
      |
      | 每帧从初始CRC=uint16(0)开始。循环一次取一个字节，把该字节乘256移到高8位，与旧CRC异或，得到
      | Merged，再交给TableStep执行查表移位。TableStep的输出成为处理下一个字节的旧CRC。
      |
      | 公式第一步是Merged=bitxor(旧CRC,当前字节×256)。整个循环结束后输出最后一次CRC，父级拆成高、
      | 低字节用于比较或发送。For Iterator中的CRC记忆是帧内累积状态，不能理解成跨帧无限累加。
      |
      | 这里用的是CRC16_Table_Reference指定的算法表，不能随意换另一种CRC表或初始值。相同字节、顺序
      | 、表和初值必须得到相同结果，双方才能校验通过。
  note: 【中文学习说明：CRC16查表法】
      | 一、大白话：把逐位算出的答案预先放进表里。
      | 收到每个字节后，用旧校验值和当前字节算一个表下标，
      | 直接查出结果，再与旧值左移一个字节后的部分异或。
      | 每字节只查一次表，不再进行8次逐位循环。
      |
      | 二、本模块一次处理15个数据字节。
      | 每帧校验值从0开始；逐字节循环仍按输入顺序执行。
      | 先将当前字节放到高八位，与旧CRC异或，
      | 再交给TableStep（查表更新）算出新CRC，
      | 记住新CRC后处理下一个字节，最后输出16位结果。
      |
      | 三、和参考工程逐项对应。
      | 参考写法：index=((旧CRC>>8) XOR 当前字节) AND 255。
      | 新CRC=表[index] XOR ((旧CRC<<8) AND 65535)。
      | 本图先合并字节再取高八位，得到完全相同的index。
      | 表为参考工程crc.c中的原始256项uint16数据，
      | 保存在模型工作区CRC16_Table_Reference中，
      | 所有CRC16模块使用同一份表，无需额外源文件。
      |
      | 四、协议规则没有改变。
      | 初值0、多项式0x1021、高位先处理、不作末尾异或。
      | 校验范围由外层选取，帧头和帧尾校验字节不随意加入。
      | 输出仍由外层拆成高、低字节，高字节在前。
      | 这里只计算CRC，是否采纳数据由外层校验比较决定。
      |
      | 五、记忆与循环要分清。
      | 外层逐字节循环在一次调用内处理整段数据，
      | 并非每处理一字节就等待一个采样周期。
      | CRC记忆块传递同一帧中上一个字节的结果；
      | 每次重新计算一帧时从0开始，不串用上一帧的结果。
      | 查表能发现传输错误，不能修复数据，也不是加密。
  Bytes（待校验字节）_616 : Inport  OutDataTypeStr=uint8
  CRC（本帧累计校验值）_618 : UnitDelay  InitialCondition=uint16(0)  SampleTime=-1  HasFrameUpgradeWarning=on
  Cast（数据类型转换）_620 : DataTypeConversion  OutDataTypeStr=uint16  RndMeth=Round
  Constant（常量）_621 : Constant  Value=256  OutDataTypeStr=uint16
  CurrentByte（当前字节）_619 : Selector  InputPortWidth=15  IndexOptions=Index vector (port)  Indices=1  OutputSizes=1
  EachByte（逐字节校验）_617 : ForIterator  ResetStates=reset  IterationLimit=15  IterationVariableDataType=uint32
  HighByte（字节移到高八位）_622 : Product  Inputs=**  SaturateOnIntegerOverflow=on  OutDataTypeStr=Inherit: Same as first input
  MergeByte（并入一个字节）_623 : simulink/Logic and Bit Operations/Bitwise Operator  logicop=XOR  UseBitMask=off  NumInputPorts=2  BitMask=bin2dec('11011001')  BitMaskRealWorld=Stored Integer
      settings: LibrarySourceBlock=|
      | hdlsllib/Logic and Bit
      | Operations/Bitwise
      | Operator
  Store_uint16（按十六位无符号数保存状态）_537120 : DataTypeConversion  Description=为反馈回路显式指定原程序的状态类型，保持原状态更新节拍。  OutDataTypeStr=uint16  RndMeth=Round
  TableStep（查表更新本字节校验） : Subsystem  Description=|
      | CRC16的一个字节怎样查表更新
      | 
      | 父级已经把当前数据字节异或进旧CRC的高8位，形成Merged。本模块把这个16位数拆成“用哪项表”和“保留哪些移位结果”两部分。
      | 
      | 先取高8位：索引=floor(Merged/256)，范围0～255。用它到CRC16_Table_Reference查表；模型Selector按零基索引取值，写成MATLAB数组下标时要用索引+1。
      | 另一条支路把Merged左移一个字节，即乘256，然后只保留低16位：移位值=bitand(uint32(Merged)×256,65535)。
      | 
      | 最后将表值与移位值按位异或：
      | 新CRC=bitxor(表值,移位值)。
      | 
      | 例如Merged=十六进制1234，高8位12用于选表项，左移并截16位后为3400，再与表项异或。宽类型uint32是为了中间计算不先溢出，并不表示输出CRC变成32位。结果回到父级，继续处理下一个数据字节。
  CRC16（本帧校验结果）_645 : Outport
  wires:
  HighByte（字节移到高八位）_622/1 -> MergeByte（并入一个字节）_623/2  "HighByte（字节移到高八位）"
  CurrentByte（当前字节）_619/1 -> Cast（数据类型转换）_620/1  "CurrentByte（当前字节）"
  Store_uint16（按十六位无符号数保存状态）_537120/1 -> CRC（本帧累计校验值）_618/1
  CRC（本帧累计校验值）_618/1 -> MergeByte（并入一个字节）_623/1  "CRC（本帧累计校验值）"
  Bytes（待校验字节）_616/1 -> CurrentByte（当前字节）_619/1  "Bytes（待校验字节）"
  EachByte（逐字节校验）_617/1 -> CurrentByte（当前字节）_619/2  "EachByte（逐字节校验）"
  TableStep（查表更新本字节校验）/1(CRC（本字节处理后的校验值）) -> Store_uint16（按十六位无符号数保存状态）_537120/1, CRC16（本帧校验结果）_645/1  "CRC16（查表更新结果）"
  Cast（数据类型转换）_620/1 -> HighByte（字节移到高八位）_622/1  "Cast（数据类型转换）"
  MergeByte（并入一个字节）_623/1 -> TableStep（查表更新本字节校验）/1(Merged（旧校验值与当前字节异或后的数）)  "Merged（旧CRC与当前字节合并值）"
  Constant（常量）_621/1 -> HighByte（字节移到高八位）_622/2  "Constant（常量）"

== system turbo_controller/COMMRead_ISM/ISM/AnalogFilter_Nc/GeneralFilter/Subsystem/Subsystem1 ==
  note: 计算低通滤波中新样本的权重
      |
      | 输入T为滤波时间常数（s），T_Sampling为采样周期（s）。输出α=T_Sampling/(T+T_Sampling)，供
      | 父级乘以本拍的新输入。
      |
      | 当前T=0.067、采样周期0.02，α=0.02/0.087≈0.229885。也就是每拍只采用约23%的新值，另外约77%
      | 由历史结果补足。时间常数越大，新值权重越小，结果越平稳但响应越慢。
      |
      | 本模块只算一个无量纲系数，不含延迟，也不直接输出温度、压力或转速。两项时间输入必须使用同一
      | 单位。
  T : Inport
      settings: AttributesFormatString=T（温度、时间或真分支输入）
  T_Sampling : Inport  Port=2
      settings: AttributesFormatString=T_Sampling（采样周期）
  Constant : Constant  OutDataTypeStr=single
      settings: AttributesFormatString=Constant（常量）
  Constant2 : Constant  OutDataTypeStr=single
      settings: AttributesFormatString=Constant2（常量2）
  Divide : Product  Inputs=*/
      settings: AttributesFormatString=Divide（除法）
  Product : Product  RndMeth=Zero
      settings: AttributesFormatString=Product（乘法）
  Product1 : Product  RndMeth=Zero
      settings: AttributesFormatString=Product1（乘法1）
  Sum : Sum  Inputs=|++
      settings: AttributesFormatString=Sum（加法求和）
  Out : Outport
      settings: AttributesFormatString=Out（输出）
  wires:
  Constant/1 -> Product/1
  T_Sampling/1 -> Product/2, Sum/2
  Product/1 -> Divide/1
  Constant2/1 -> Product1/1
  T/1 -> Product1/2
  Product1/1 -> Sum/1
  Sum/1 -> Divide/2
  Divide/1 -> Out/1

== system turbo_controller/COMMRead_ISM/ISM/AnalogFilter_Nc/GeneralFilter/Subsystem/Subsystem2 ==
  note: 计算低通滤波中历史结果的权重
      |
      | 输入T为时间常数，T_Sampling为采样周期，两者都用s。输出β=T/(T+T_Sampling)，供父级乘以上一
      | 次滤波结果。
      |
      | 当前T=0.067、采样周期0.02，β≈0.770115；与另一支路新样本权重α≈0.229885相加为1。这样常值
      | 输入最终会稳定在原值，不会因为反复相加而不断放大。
      |
      | 本模块只计算系数，历史结果由父级延迟块保存。若把20 ms误传成20 s，权重和滤波速度都会完全改
      | 变，因此父级先将Ts_ms除以1000。
  T : Inport
      settings: AttributesFormatString=T（温度、时间或真分支输入）
  T_Sampling : Inport  Port=2
      settings: AttributesFormatString=T_Sampling（采样周期）
  Constant : Constant  OutDataTypeStr=single
      settings: AttributesFormatString=Constant（常量）
  Constant2 : Constant  OutDataTypeStr=single
      settings: AttributesFormatString=Constant2（常量2）
  Divide : Product  Inputs=*/
      settings: AttributesFormatString=Divide（除法）
  Product : Product  RndMeth=Zero
      settings: AttributesFormatString=Product（乘法）
  Product1 : Product  RndMeth=Zero
      settings: AttributesFormatString=Product1（乘法1）
  Sum : Sum  Inputs=|++
      settings: AttributesFormatString=Sum（加法求和）
  Out : Outport
      settings: AttributesFormatString=Out（输出）
  wires:
  Constant/1 -> Product/1
  T/1 -> Product/2, Product1/2
  Product/1 -> Divide/1
  Constant2/1 -> Product1/1
  Product1/1 -> Sum/1
  T_Sampling/1 -> Sum/2
  Sum/1 -> Divide/2
  Divide/1 -> Out/1

== system turbo_controller/BoardInput_输入换算与协议解析/In02_Motor（电机反馈解析）/Receive（逐字节组帧与保持有效结果）_235/Step03_收齐且校验通过才接受/Verify（完整帧校验）_218/CRC16（循环冗余校验）_202/TableStep（查表更新本字节校验） ==
  note: CRC16的一个字节怎样查表更新
      |
      | 父级已经把当前数据字节异或进旧CRC的高8位，形成Merged。本模块把这个16位数拆成“用哪项表”和
      | “保留哪些移位结果”两部分。
      |
      | 先取高8位：索引=floor(Merged/256)，范围0～255。用它到CRC16_Table_Reference查表；模型Select
      | or按零基索引取值，写成MATLAB数组下标时要用索引+1。
      | 另一条支路把Merged左移一个字节，即乘256，然后只保留低16位：移位值=bitand(uint32(Merged)×25
      | 6,65535)。
      |
      | 最后将表值与移位值按位异或：
      | 新CRC=bitxor(表值,移位值)。
      |
      | 例如Merged=十六进制1234，高8位12用于选表项，左移并截16位后为3400，再与表项异或。宽类型uint
      | 32是为了中间计算不先溢出，并不表示输出CRC变成32位。结果回到父级，继续处理下一个数据字节。
  Merged（旧校验值与当前字节异或后的数） : Inport  OutDataTypeStr=uint16
  CRC16Table（参考工程原始二百五十六项表） : Constant  Value=CRC16_Table_Reference  OutDataTypeStr=uint16
  Divisor（高字节换算除数） : Constant  Value=256  OutDataTypeStr=double
  Exact（转双精度做精确除法） : DataTypeConversion  OutDataTypeStr=double  SaturateOnIntegerOverflow=off  RndMeth=Floor
  HighByte（除二百五十六取高字节） : Product  Inputs=*/  OutDataTypeStr=double
  Index（向下取整得到零至二百五十五） : DataTypeConversion  OutDataTypeStr=uint32  RndMeth=Floor
  LeftByte（左移一个字节） : Product  Inputs=**  OutDataTypeStr=uint32  SaturateOnIntegerOverflow=on
  Lookup（按零基索引读取校验表） : Selector  IndexMode=Zero-based  InputPortWidth=256  IndexOptions=Index vector (port)  Indices=1  OutputSizes=1
  Mask16（保留低十六位） : Constant  Value=65535  OutDataTypeStr=uint32
  Shift16（移位结果转十六位） : DataTypeConversion  OutDataTypeStr=uint16  SaturateOnIntegerOverflow=off  RndMeth=Floor
  ShiftBase（一个字节的移位系数） : Constant  Value=256  OutDataTypeStr=uint32
  Update（查表值与移位结果异或） : simulink/Logic and Bit Operations/Bitwise Operator  logicop=XOR  UseBitMask=off  NumInputPorts=2  BitMask=bin2dec('11011001')  BitMaskRealWorld=Stored Integer
      settings: LibrarySourceBlock=|
      | hdlsllib/Logic and Bit
      | Operations/Bitwise
      | Operator
  Wide（转三十二位防止移位溢出） : DataTypeConversion  OutDataTypeStr=uint32  SaturateOnIntegerOverflow=off  RndMeth=Floor
  Wrap16（截取左移后的低十六位） : simulink/Logic and Bit Operations/Bitwise Operator  logicop=AND  UseBitMask=off  NumInputPorts=2  BitMask=bin2dec('11011001')  BitMaskRealWorld=Stored Integer
      settings: LibrarySourceBlock=|
      | hdlsllib/Logic and Bit
      | Operations/Bitwise
      | Operator
  CRC（本字节处理后的校验值） : Outport
  wires:
  Merged（旧校验值与当前字节异或后的数）/1 -> Exact（转双精度做精确除法）/1, Wide（转三十二位防止移位溢出）/1
  Wide（转三十二位防止移位溢出）/1 -> LeftByte（左移一个字节）/1
  ShiftBase（一个字节的移位系数）/1 -> LeftByte（左移一个字节）/2
  LeftByte（左移一个字节）/1 -> Wrap16（截取左移后的低十六位）/1
  Mask16（保留低十六位）/1 -> Wrap16（截取左移后的低十六位）/2
  Wrap16（截取左移后的低十六位）/1 -> Shift16（移位结果转十六位）/1
  Exact（转双精度做精确除法）/1 -> HighByte（除二百五十六取高字节）/1
  Divisor（高字节换算除数）/1 -> HighByte（除二百五十六取高字节）/2
  HighByte（除二百五十六取高字节）/1 -> Index（向下取整得到零至二百五十五）/1
  CRC16Table（参考工程原始二百五十六项表）/1 -> Lookup（按零基索引读取校验表）/1
  Index（向下取整得到零至二百五十五）/1 -> Lookup（按零基索引读取校验表）/2
  Lookup（按零基索引读取校验表）/1 -> Update（查表值与移位结果异或）/1
  Shift16（移位结果转十六位）/1 -> Update（查表值与移位结果异或）/2
  Update（查表值与移位结果异或）/1 -> CRC（本字节处理后的校验值）/1
